simulink model "sim_conv"  (Simulink 7.4)
settings: Solver=ode45  StartTime=0.0  StopTime=1  RelTol=1e-3
undefined symbols (not defined in the file or in its folder): serial
libraries: instrumentlib x3, powerlib x1
settings Model: Creator=Danilo  LastModifiedBy=Danilo

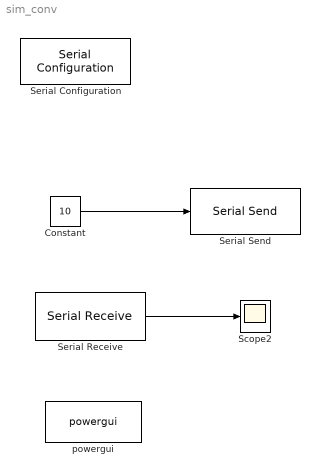
== system sim_conv ==
  Constant : Constant  Value=10  OutDataType=fixdt(1, 16)  OutScaling=2^0  SampleTime=1e-3
  Scope2 : Scope
      settings: TimeRange=0.03563218390804598  YMin=10  YMax=10
  Serial Configuration : instrumentlib/Serial Configuration  Priority=-200000  DialogController=instrumentcreatedialog  DialogControllerArgs=DataTag0  ComPortMenu=COM4  ComPort=COM4  ObjConstructor=serial('COM4');  BaudRate=9600  DataBits=8  Parity=none  StopBits=1  FlowControl=hardware  Timeout=10  ByteOrder=LittleEndian
  Serial Receive : instrumentlib/Serial Receive  DialogController=instrumentcreatedialog  DialogControllerArgs=DataTag1  ComPortMenu=COM4  ComPort=COM4  ObjConstructor=serial('COM4');  Terminator=<none>  DataSize=[1 1]  DataType=double  EnableBlockingMode=on  ActionDataUnavailable=Output last received value  CustomValue=2  SampleTime=0.001
  Serial Send : instrumentlib/Serial Send  DialogController=instrumentcreatedialog  DialogControllerArgs=DataTag2  ComPortMenu=COM4  ComPort=COM4  ObjConstructor=serial('COM4');  Terminator=<none>  EnableBlockingMode=on
  powergui : powerlib/powergui  Priority=1  SystemSampleTime=-1  SimulationMode=Discrete  SampleTime=1e-3  frequency=60  SPID=off  DisableSnubberDevices=off  DisableRonSwitches=off  DisableVfSwitches=off  SwTol=0  Interpol=off  frequencyindice=0  echomessages=off  HookPort=off  DisplayEquations=off  FunctionMessages=off  EnableUseOfTLC=off  x0status=blocks  RestoreLinks=warning  Frange=[0:2:500]  Ylog=off  Xlog=on  ShowGrid=off  save=off  variable=ZData  ZoomFFT=on  StartTime=0.0  cycles=1  DisplayStyle=1  fundamental=60  FreqAxis=off  MaxFrequency=1000  frequencyindicesteady=1  RmsSteady=1  display=off  Ts=0  methode=off
  wires:
  Serial Receive/1 -> Scope2/1
  Constant/1 -> Serial Send/1
